simulink model "heli_q8_final"  (R2020b)
settings: Solver=ode1  StartTime=0.0  StopTime=inf  FixedStep=0.002  RelTol=1e-3  EnableMultiTasking=on
PostLoadFcn:
  | qc_set_target_type(getConfigSet(bdroot, 'QUARC Default Target Configuration'));
undefined symbols (not defined in the file or in its folder): A_d, A_obs, B_d, B_obs, C, C_d, elevation_offset, F, HIL, Joystick_gain_x, Joystick_gain_y, K, Kpd, Kpp, L, Q_d, qc_get_step_size, R_flying, V_s0
libraries: quarc_library x34, simulink x7, pid_lib x1
(part 1 of 2)
settings Model: SimulationMode=external  ExtModeTrigDuration=600000  Creator=Rchan  LastModifiedBy=wiktorjr
settings SolverCC: PositivePriorityOrder=on
settings DataIOCC: LimitDataPoints=on  SaveFormat=Array  SignalLoggingSaveFormat=ModelDataLogs  ReturnWorkspaceOutputs=off
settings OptimizationCC: ExpressionDepthLimit=2147483647  InitFltsAndDblsToZero=on  LifeSpan=inf
settings DebuggingCC: SaveWithParameterizedLinksMsg=none  UnderspecifiedInitializationDetection=Classic  MergeDetectMultiDrivingBlocksExec=none  SolverPrmCheckMsg=warning  MultiTaskDSMMsg=warning  MultiTaskCondExecSysMsg=none  FcnCallInpInsideContextMsg=warning  AllowSymbolicDim=off  StateNameClashWarn=warning  SFUnexpectedBacktrackingDiag=warning  SFNoUnconditionalDefaultTransitionDiag=warning  SFExecutionAtInitializationDiag=none  ArithmeticOperatorsInVariantConditions=warning
settings HardwareCC: ProdBitPerPointer=32  ProdBitPerSizeT=32  ProdBitPerPtrDiffT=32  ProdLargestAtomicFloat=None  ProdIntDivRoundTo=Undefined  ProdEndianess=Unspecified  ProdWordSize=32  ProdHWDeviceType=32-bit Generic
settings ModelReferenceCC: PropagateSignalLabelsOutOfModel=off
settings SFSimCC: SimUseLocalCustomCode=off  CustomCodeUndefinedFunction=UseInterfaceOnly
settings RTWCC: Description=QUARC Win64 Target  SystemTargetFile=quarc_win64.tlc  TemplateMakefile=quarc_default_tmf  RTWUseLocalCustomCode=off
settings CodeAppCC: StateflowObjectComments=on
settings GRTTargetCC: TargetLangStandard=C89/C90 (ANSI)  ParMdlRefBuildCompliant=off  CompOptLevelCompliant=off  CombineOutputUpdateFcns=off  MatFileLogging=off  GRTInterface=on  UseToolchainInfoCompliant=off  ExtMode=on  ExtModeMexFile=quarc_comm
settings ConfigComp: CovMetricSettings=dw  CovSaveCumulativeToWorkspaceVar=on  CovSaveSingleToWorkspaceVar=on  CovExternalEMLEnable=off  CovSFcnEnable=off

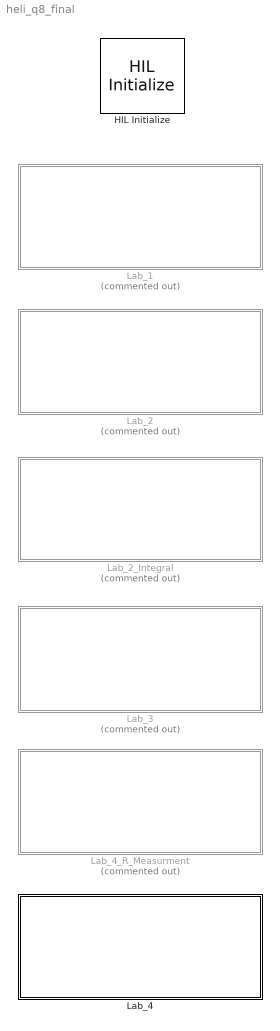
== system heli_q8_final ==
  HIL Initialize : quarc_library/Data Acquisition/Generic/Configuration/HIL Initialize  Priority=-99  object_name=HIL-1  board_type=q8_usb  board_number=0  board_options=update_rate=normal;decimation=1  exclusive=off  active=off  hardware_clocks=[0:2]  clock_modes=[]  initial_clock_frequencies=[]  set_clock_params_at_start=off  set_clock_params_at_switch_in=off  set_clock_frequencies_at_start=off  set_clock_frequencies_at_switch_in=off  analog_input_channels=[0:7]  analog_input_configurations=[]  analog_input_maximums=10  analog_input_minimums=-10  set_analog_input_params_at_start=on  set_analog_input_params_at_switch_in=off  analog_output_channels=[0:7]  analog_output_maximums=10  analog_output_minimums=-10  initial_analog_outputs=[0]  final_analog_outputs=[0]  watchdog_analog_outputs=0  set_analog_output_params_at_start=on  set_analog_output_params_at_switch_in=off  set_analog_outputs_at_start=on  set_analog_outputs_at_switch_in=off  set_analog_outputs_at_terminate=on  set_analog_outputs_at_switch_out=off  set_analog_outputs_on_watchdog=off  digital_input_channels=[]  digital_output_channels=[]  digital_output_configuration=[]  initial_digital_outputs=[1]  final_digital_outputs=[1]  watchdog_digital_outputs=[1]  set_digital_output_params_at_start=off  set_digital_output_params_at_switch_in=off  set_digital_outputs_at_start=on  set_digital_outputs_at_switch_in=off  set_digital_outputs_at_terminate=on  set_digital_outputs_at_switch_out=off  set_digital_outputs_on_watchdog=off  encoder_channels=[0:7]  quadrature=[4]  encoder_filter_frequency=[]  initial_encoder_counts=[0]  set_encoder_params_at_start=on  set_encoder_params_at_switch_in=off  set_encoder_counts_at_start=on  set_encoder_counts_at_switch_in=off  pwm_channels=[0:7]  pwm_modes=0  pwm_frequency=99.532799999999995e6/4095  pwm_configuration=[0]  pwm_alignment=[0]  pwm_polarity=[1]  pwm_leading_deadband=[0]  pwm_trailing_deadband=[0]  initial_pwm_outputs=[0]  final_pwm_outputs=[0]  watchdog_pwm_outputs=[0]  set_pwm_params_at_start=on  set_pwm_params_at_switch_in=off  set_pwm_outputs_at_start=on  set_pwm_outputs_at_switch_in=off  set_pwm_outputs_at_terminate=on  set_pwm_outputs_at_switch_out=off  set_pwm_outputs_on_watchdog=off  other_output_channels=[]  initial_other_outputs=[]  final_other_outputs=[]  watchdog_other_outputs=[]  set_other_outputs_at_start=off  set_other_outputs_at_switch_in=off  set_other_outputs_at_terminate=off  set_other_outputs_at_switch_out=off  set_other_outputs_on_watchdog=off
  Lab_1 : Subsystem  Commented=on
  Lab_2 : Subsystem  Commented=on
  Lab_2_Integral : Subsystem  Commented=on
  Lab_3 : Subsystem  Commented=on
  Lab_4 : Subsystem
  Lab_4_R_Measurment : Subsystem  Commented=on

== system heli_q8_final/Lab_1 ==
  note: Pitch test signal
  note: Elevation test signal
  Constant2 : Constant  Value=0
  Constant3 : Constant  Value=0.5
  Conversion : Subsystem
  Demux : Demux  Outputs=6
  Demux1 : Demux  Outputs=8
  Elevation controller : Subsystem
  Heli 3D : Subsystem
  Joystick : Subsystem
  Manual Switch2 : ManualSwitch
  Manual Switch3 : ManualSwitch  CurrentSetting=0
  Mux : Mux  Inputs=6
  Mux1 : Mux  Inputs=3
  Pitch controller : Subsystem
  Pulse Generator : DiscretePulseGenerator  PulseType=Time based  Amplitude=-1  Period=40  PulseWidth=50
  Ramp1 : simulink/Sources/Ramp  slope=0.05  start=0  InitialOutput=-0.5
  Ramp3 : simulink/Sources/Ramp  slope=0.1  start=45  InitialOutput=0
  Saturation : Saturate  UpperLimit=0
  Saturation2 : Saturate  LowerLimit=0
  Scope : Scope  NumInputPorts=4
  Step1 : Step  Time=15  SampleTime=0
  Step4 : Step  Time=40  SampleTime=0
  Sum1 : Sum  Inputs=+-|
  Sum4 : Sum  Inputs=+|-
  Sum5 : Sum  Inputs=+|+
  Switch : Switch  Criteria=u2 > Threshold
  To File : ToFile  Filename=Test.mat
  wires:
  Demux/4 -> Pitch controller/3(p~dot [rad/s])  "p~dot"
  Mux/1 -> Mux1/1, Demux/1
  Manual Switch2/1 -> Mux1/2, Pitch controller/1(p~c [rad])  "p_c"
  Elevation controller/1(V~s [V]) -> Conversion/2(Vs [V])
  Heli 3D/2(Travel rate [rad/s]) -> Mux/2  "lambda~_dot"
  Pitch controller/1(V~d [V]) -> Conversion/1(Vd [V])
  Heli 3D/6(Elevation rate [rad/s]) -> Mux/6  "e~dot"
  Demux/3 -> Pitch controller/2(p~ [rad])  "p~"
  Demux/6 -> Elevation controller/2(e~dot [rad/s])  "e~dot"
  Heli 3D/1(Travel [rad]) -> Mux/1  "lambda~"
  Conversion/2(Vb [V]) -> Heli 3D/2(Vb [V])
  Demux/5 -> Elevation controller/1(e~ [rad])  "e~"
  Heli 3D/5(Elevation [rad]) -> Mux/5  "e~"
  Heli 3D/3(Pitch [rad]) -> Mux/3  "p~"
  Heli 3D/4(Pitch rate [rad/s]) -> Mux/4  "p~dot"
  Conversion/1(Vf [V]) -> Heli 3D/1(Vf [V])
  Sum1/1 -> Manual Switch3/2
  Manual Switch3/1 -> Mux1/3, Elevation controller/3(e~c [rad])  "e_c"
  Sum5/1 -> Switch/1
  Joystick/2(Y) -> Manual Switch3/1  "e_c"
  Sum4/1 -> Switch/2
  Step4/1 -> Sum4/2
  Step1/1 -> Sum4/1
  Constant3/1 -> Sum5/2
  Joystick/1(X) -> Manual Switch2/2  "p_c"
  Switch/1 -> Manual Switch2/1
  Pulse Generator/1 -> Sum5/1
  Constant2/1 -> Switch/3
  Mux1/1 -> Demux1/1, To File/1
  Demux1/7 -> Scope/3  "p_c"
  Demux1/8 -> Scope/4  "e_c"
  Demux1/3 -> Scope/1  "p~"
  Demux1/5 -> Scope/2  "e~"
  Ramp1/1 -> Saturation/1
  Ramp3/1 -> Saturation2/1
  Saturation/1 -> Sum1/1
  Saturation2/1 -> Sum1/2

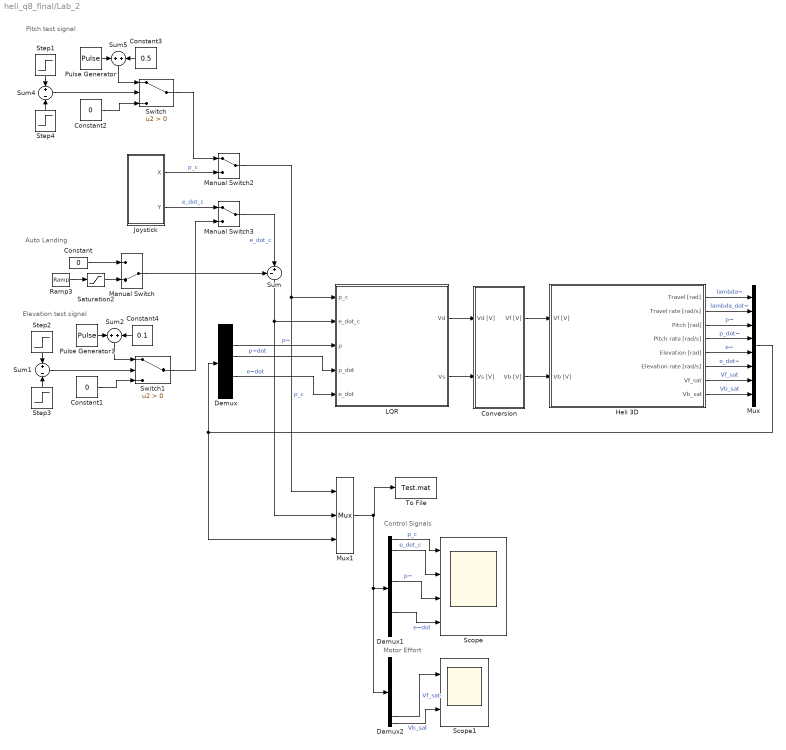
== system heli_q8_final/Lab_2 ==
  note: Auto Landing
  note: Motor Effort
  note: Control Signals
  note: Elevation test signal
  note: Pitch test signal
  Constant : Constant  Value=0
  Constant1 : Constant  Value=0
  Constant2 : Constant  Value=0
  Constant3 : Constant  Value=0.5
  Constant4 : Constant  Value=0.1
  Conversion : Subsystem
  Demux : Demux  Outputs=8
  Demux1 : Demux  Outputs=10
  Demux2 : Demux  Outputs=10
  Heli 3D : Subsystem
  Joystick : Subsystem
  LQR : Subsystem
  Manual Switch : ManualSwitch  CurrentSetting=0
  Manual Switch2 : ManualSwitch
  Manual Switch3 : ManualSwitch
  Mux : Mux  Inputs=8
  Mux1 : Mux  Inputs=3
  Pulse Generator : DiscretePulseGenerator  PulseType=Time based  Amplitude=-1  Period=15  PulseWidth=50
  Pulse Generator1 : DiscretePulseGenerator  PulseType=Time based  Amplitude=-0.2  Period=10  PulseWidth=50
  Ramp3 : simulink/Sources/Ramp  slope=0.15  start=45  InitialOutput=0
  Saturation2 : Saturate  UpperLimit=1  LowerLimit=0
  Scope : Scope  NumInputPorts=4
  Scope1 : Scope  NumInputPorts=2
  Step1 : Step  Time=15  SampleTime=0
  Step2 : Step  Time=15  SampleTime=0
  Step3 : Step  Time=40  SampleTime=0
  Step4 : Step  Time=40  SampleTime=0
  Sum : Sum  Inputs=-+|
  Sum1 : Sum  Inputs=+|-
  Sum2 : Sum  Inputs=+|+
  Sum4 : Sum  Inputs=+|-
  Sum5 : Sum  Inputs=+|+
  Switch : Switch  Criteria=u2 > Threshold
  Switch1 : Switch  Criteria=u2 > Threshold
  To File : ToFile  Filename=Test.mat
  wires:
  Heli 3D/4(Pitch rate [rad/s]) -> Mux/4  "p_dot~"
  Demux/6 -> LQR/5(e_dot)  "e~dot"
  Demux/3 -> LQR/3(p)  "p~"
  Heli 3D/3(Pitch [rad]) -> Mux/3  "p~"
  Manual Switch2/1 -> LQR/1(p_c), Mux1/1  "p_c"
  Manual Switch3/1 -> Sum/2  "e_dot_c"
  Mux/1 -> Mux1/3, Demux/1
  Demux/4 -> LQR/4(p_dot)  "p~dot"
  Heli 3D/5(Elevation [rad]) -> Mux/5  "e~"
  Conversion/1(Vf [V]) -> Heli 3D/1(Vf [V])
  Heli 3D/6(Elevation rate [rad/s]) -> Mux/6  "e_dot~"
  Heli 3D/1(Travel [rad]) -> Mux/1  "lambda~"
  Heli 3D/2(Travel rate [rad/s]) -> Mux/2  "lambda_dot~"
  Conversion/2(Vb [V]) -> Heli 3D/2(Vb [V])
  LQR/1(Vd) -> Conversion/1(Vd [V])
  LQR/2(Vs) -> Conversion/2(Vs [V])
  Joystick/1(X) -> Manual Switch2/2  "p_c"
  Step4/1 -> Sum4/2
  Pulse Generator/1 -> Sum5/1
  Constant3/1 -> Sum5/2
  Sum4/1 -> Switch/2
  Sum5/1 -> Switch/1
  Step1/1 -> Sum4/1
  Constant2/1 -> Switch/3
  Switch/1 -> Manual Switch2/1
  Joystick/2(Y) -> Manual Switch3/1  "e_dot_c"
  Heli 3D/7(Vf_sat) -> Mux/7  "Vf_sat"
  Heli 3D/8(Vb_sat) -> Mux/8  "Vb_sat"
  Mux1/1 -> Demux2/1, Demux1/1, To File/1
  Demux1/1 -> Scope/1  "p_c"
  Demux1/2 -> Scope/2  "e_dot_c"
  Demux1/5 -> Scope/3  "p~"
  Demux1/8 -> Scope/4  "e~dot"
  Demux2/9 -> Scope1/1  "Vf_sat"
  Demux2/10 -> Scope1/2  "Vb_sat"
  Step2/1 -> Sum1/1
  Sum2/1 -> Switch1/1
  Constant1/1 -> Switch1/3
  Pulse Generator1/1 -> Sum2/1
  Constant4/1 -> Sum2/2
  Step3/1 -> Sum1/2
  Sum1/1 -> Switch1/2
  Ramp3/1 -> Saturation2/1
  Switch1/1 -> Manual Switch3/2
  Saturation2/1 -> Manual Switch/2
  Constant/1 -> Manual Switch/1
  Manual Switch/1 -> Sum/1
  Sum/1 -> Mux1/2, LQR/2(e_dot_c)

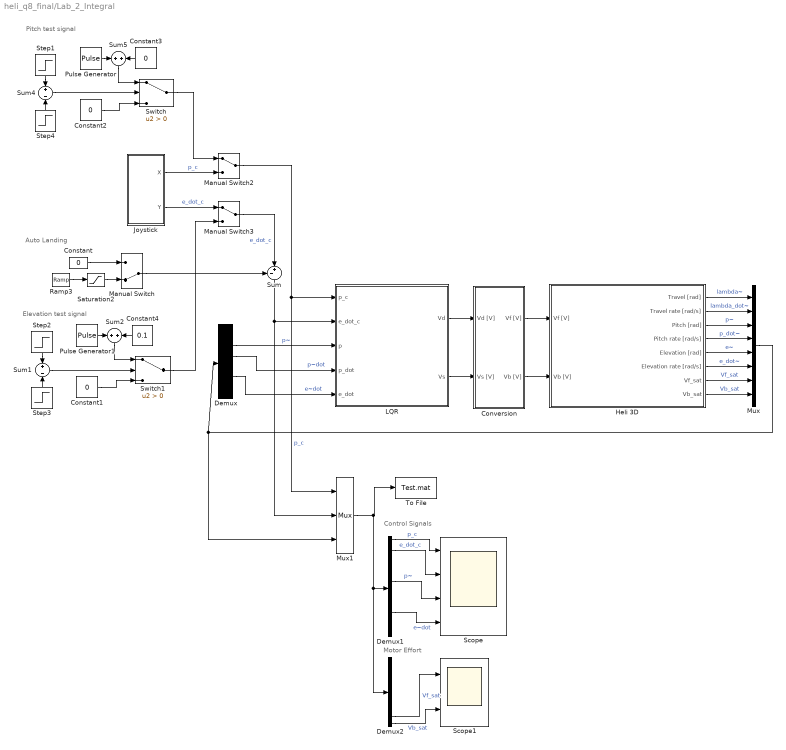
== system heli_q8_final/Lab_2_Integral ==
  note: Auto Landing
  note: Elevation test signal
  note: Motor Effort
  note: Pitch test signal
  note: Control Signals
  Constant{,1..3} (4 alike) : Constant  Value=0
  Constant4 : Constant  Value=0.1
  Conversion : Subsystem
  Demux : Demux  Outputs=8
  Demux1 : Demux  Outputs=10
  Demux2 : Demux  Outputs=10
  Heli 3D : Subsystem
  Joystick : Subsystem
  LQR : Subsystem
  Manual Switch : ManualSwitch  CurrentSetting=0
  Manual Switch2 : ManualSwitch
  Manual Switch3 : ManualSwitch
  Mux : Mux  Inputs=8
  Mux1 : Mux  Inputs=3
  Pulse Generator : DiscretePulseGenerator  PulseType=Time based  Amplitude=-0.5  Period=15  PulseWidth=50  PhaseDelay=-10
  Pulse Generator1 : DiscretePulseGenerator  PulseType=Time based  Amplitude=-0.2  Period=10  PulseWidth=50
  Ramp3 : simulink/Sources/Ramp  slope=0.15  start=45  InitialOutput=0
  Saturation2 : Saturate  UpperLimit=1  LowerLimit=0
  Scope : Scope  NumInputPorts=4
  Scope1 : Scope  NumInputPorts=2
  Step1 : Step  Time=15  SampleTime=0
  Step2 : Step  Time=15  SampleTime=0
  Step3 : Step  Time=40  SampleTime=0
  Step4 : Step  Time=40  SampleTime=0
  Sum : Sum  Inputs=-+|
  Sum1 : Sum  Inputs=+|-
  Sum2 : Sum  Inputs=+|+
  Sum4 : Sum  Inputs=+|-
  Sum5 : Sum  Inputs=+|+
  Switch : Switch  Criteria=u2 > Threshold
  Switch1 : Switch  Criteria=u2 > Threshold
  To File : ToFile  Filename=Test.mat
  wires:
  Sum/1 -> Mux1/2, LQR/2(e_dot_c)
  Constant4/1 -> Sum2/2
  Ramp3/1 -> Saturation2/1
  Constant2/1 -> Switch/3
  Demux/3 -> LQR/3(p)  "p~"
  Step3/1 -> Sum1/2
  Demux1/1 -> Scope/1  "p_c"
  Switch1/1 -> Manual Switch3/2
  Constant/1 -> Manual Switch/1
  Heli 3D/5(Elevation [rad]) -> Mux/5  "e~"
  Mux/1 -> Mux1/3, Demux/1
  Demux1/2 -> Scope/2  "e_dot_c"
  Demux1/8 -> Scope/4  "e~dot"
  Demux2/9 -> Scope1/1  "Vf_sat"
  Demux2/10 -> Scope1/2  "Vb_sat"
  Sum1/1 -> Switch1/2
  Sum4/1 -> Switch/2
  Pulse Generator1/1 -> Sum2/1
  Manual Switch/1 -> Sum/1
  Heli 3D/4(Pitch rate [rad/s]) -> Mux/4  "p_dot~"
  Heli 3D/8(Vb_sat) -> Mux/8  "Vb_sat"
  Constant1/1 -> Switch1/3
  Step2/1 -> Sum1/1
  Switch/1 -> Manual Switch2/1
  LQR/2(Vs) -> Conversion/2(Vs [V])
  Step4/1 -> Sum4/2
  Pulse Generator/1 -> Sum5/1
  Manual Switch2/1 -> Mux1/1, LQR/1(p_c)  "p_c"
  Saturation2/1 -> Manual Switch/2
  Mux1/1 -> Demux2/1, Demux1/1, To File/1
  Demux1/5 -> Scope/3  "p~"
  Constant3/1 -> Sum5/2
  Sum2/1 -> Switch1/1
  Heli 3D/2(Travel rate [rad/s]) -> Mux/2  "lambda_dot~"
  Sum5/1 -> Switch/1
  Manual Switch3/1 -> Sum/2  "e_dot_c"
  Step1/1 -> Sum4/1
  Heli 3D/1(Travel [rad]) -> Mux/1  "lambda~"
  Joystick/1(X) -> Manual Switch2/2  "p_c"
  Demux/4 -> LQR/4(p_dot)  "p~dot"
  Joystick/2(Y) -> Manual Switch3/1  "e_dot_c"
  Heli 3D/7(Vf_sat) -> Mux/7  "Vf_sat"
  LQR/1(Vd) -> Conversion/1(Vd [V])
  Heli 3D/6(Elevation rate [rad/s]) -> Mux/6  "e_dot~"
  Heli 3D/3(Pitch [rad]) -> Mux/3  "p~"
  Demux/6 -> LQR/5(e_dot)  "e~dot"
  Conversion/2(Vb [V]) -> Heli 3D/2(Vb [V])
  Conversion/1(Vf [V]) -> Heli 3D/1(Vf [V])

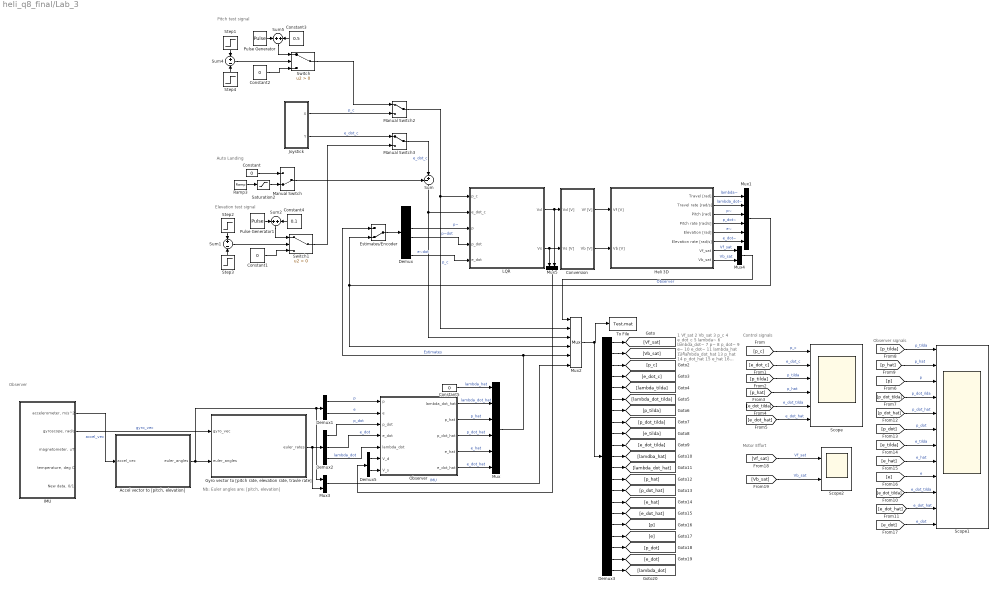
== system heli_q8_final/Lab_3 ==
  note: Motor Effort
  note: Control signals
  note: 1   Vf_sat
      | 2   Vb_sat
      | 3   p_c
      | 4   e_dot_c
      | 5   lambda~
      | 6   lambda_dot~
      | 7   p~
      | 8   p_dot~
      | 9   e~
      | 10 e_dot~
      | 11 lambda_hat
      | 12 lambda_dot_hat
      | 13 p_hat
      | 14 p_dot_hat
      | 15 e_hat
      | 16 e_dot_hat
      | 17 p
      | 18 e
      | 19 p_dot
      | 20 e_dot
      | 21 lambda_dot
  note: Observer
  note: Nb: Euler angles are: [pitch, elevation]
  note: Pitch test signal
  note: Elevation test signal
  note: Auto Landing
  note: Observer signals
  "Accel vector to [pitch, elevation]" : MATLAB Function  TreatAsAtomicUnit=on
  Constant{,1..2,5} (4 alike) : Constant  Value=0
  Constant3 : Constant  Value=0.5
  Constant4 : Constant  Value=0.1
  Conversion : Subsystem
  Demux : Demux  Outputs=6
  Demux1 : Demux  Outputs=2
  Demux2 : Demux  Outputs=3
  Demux3 : Demux  Outputs=21
  Demux5 : Demux  Outputs=2
  Estimates/Encoder : ManualSwitch  CurrentSetting=0
  "Gyro vector to [pitch rate, elevation rate, travle rate]" : MATLAB Function  TreatAsAtomicUnit=on
  Heli 3D : Subsystem
  IMU : Subsystem
  Joystick : Subsystem
  LQR : Subsystem
  Manual Switch : ManualSwitch  CurrentSetting=0
  Manual Switch2 : ManualSwitch
  Manual Switch3 : ManualSwitch
  Mux : Mux  Inputs=6
  Mux1 : Mux  Inputs=6
  Mux2 : Mux  Inputs=6
  Mux3 : Mux  Inputs=2
  Mux4 : Mux  Inputs=2
  Mux5 : Mux  Inputs=2
  Observer : Subsystem
  Pulse Generator : DiscretePulseGenerator  PulseType=Time based  Amplitude=-1  Period=15  PulseWidth=50  PhaseDelay=-10
  Pulse Generator1 : DiscretePulseGenerator  PulseType=Time based  Amplitude=-0.2  Period=10  PulseWidth=50
  Ramp3 : simulink/Sources/Ramp  slope=0.15  start=45  InitialOutput=0
  Saturation2 : Saturate  UpperLimit=1  LowerLimit=0
  Scope : Scope  NumInputPorts=6
  Scope1 : Scope  NumInputPorts=12
  Scope2 : Scope  NumInputPorts=2
  Step1 : Step  Time=15  SampleTime=0
  Step2 : Step  Time=15  SampleTime=0
  Step3 : Step  Time=40  SampleTime=0
  Step4 : Step  Time=40  SampleTime=0
  Sum : Sum  Inputs=-+|
  Sum1 : Sum  Inputs=+|-
  Sum2 : Sum  Inputs=+|+
  Sum4 : Sum  Inputs=+|-
  Sum5 : Sum  Inputs=+|+
  Switch : Switch  Criteria=u2 > Threshold
  Switch1 : Switch  Criteria=u2 > Threshold
  To File : ToFile  Filename=Test.mat
  wires:
  Demux2/1 -> Observer/3(p_dot)  "p_dot"
  "Gyro vector to [pitch rate, elevation rate, travle rate]"/1(euler_rates) -> Mux3/2, Demux2/1
  "Accel vector to [pitch, elevation]"/1(euler_angles) -> Mux3/1, Demux1/1, "Gyro vector to [pitch rate, elevation rate, travle rate]"/2(euler_angles)
  Demux2/2 -> Observer/4(e_dot)  "e_dot"
  Demux2/3 -> Observer/5(lambda_dot)  "lambda_dot"
  Demux1/2 -> Observer/2(e)  "e"
  IMU/2("gyroscope, rad/s") -> "Gyro vector to [pitch rate, elevation rate, travle rate]"/1(gyro_vec)  "gyro_vec"
  Demux1/1 -> Observer/1(p)  "p"
  IMU/1("accelerometer, m/s^2") -> "Accel vector to [pitch, elevation]"/1(accel_vec)  "accel_vec"
  Step3/1 -> Sum1/2
  Heli 3D/3(Pitch [rad]) -> Mux1/3  "p~"
  Heli 3D/7(Vf_sat) -> Mux4/1  "Vf_sat"
  Joystick/1(X) -> Manual Switch2/2  "p_c"
  Constant3/1 -> Sum5/2
  Sum5/1 -> Switch/1
  Manual Switch3/1 -> Sum/2  "e_dot_c"
  Sum2/1 -> Switch1/1
  Saturation2/1 -> Manual Switch/2
  Mux2/1 -> Demux3/1, To File/1
  Manual Switch2/1 -> Mux2/2, LQR/1(p_c)  "p_c"
  Pulse Generator/1 -> Sum5/1
  Step1/1 -> Sum4/1
  Step4/1 -> Sum4/2
  Heli 3D/4(Pitch rate [rad/s]) -> Mux1/4  "p_dot~"
  Step2/1 -> Sum1/1
  Constant1/1 -> Switch1/3
  Pulse Generator1/1 -> Sum2/1
  Heli 3D/1(Travel [rad]) -> Mux1/1  "lambda~"
  Switch/1 -> Manual Switch2/1
  Sum4/1 -> Switch/2
  Manual Switch/1 -> Sum/1
  Mux1/1 -> Estimates/Encoder/2, Mux2/4  "Observer"
  Heli 3D/2(Travel rate [rad/s]) -> Mux1/2  "lambda_dot~"
  Switch1/1 -> Manual Switch3/2
  Conversion/2(Vb [V]) -> Heli 3D/2(Vb [V])
  Heli 3D/5(Elevation [rad]) -> Mux1/5  "e~"
  Demux/3 -> LQR/3(p)  "p~"
  Constant4/1 -> Sum2/2
  Constant2/1 -> Switch/3
  Ramp3/1 -> Saturation2/1
  Sum/1 -> Mux2/3, LQR/2(e_dot_c)
  Heli 3D/8(Vb_sat) -> Mux4/2  "Vb_sat"
  Joystick/2(Y) -> Manual Switch3/1  "e_dot_c"
  LQR/2(Vs) -> Conversion/2(Vs [V]), Mux5/1
  Constant/1 -> Manual Switch/1
  Sum1/1 -> Switch1/2
  Heli 3D/6(Elevation rate [rad/s]) -> Mux1/6  "e_dot~"
  Demux/6 -> LQR/5(e_dot)  "e~dot"
  Demux/4 -> LQR/4(p_dot)  "p~dot"
  LQR/1(Vd) -> Conversion/1(Vd [V]), Mux5/2
  Conversion/1(Vf [V]) -> Heli 3D/1(Vf [V])
  Mux/1 -> Estimates/Encoder/1, Mux2/5  "Estimates"
  Mux3/1 -> Mux2/6  "IMU"
  Mux4/1 -> Mux2/1
  Constant5/1 -> Mux/1  "lambda_hat"
  Observer/1(lambda_dot_hat) -> Mux/2  "lambda_dot_hat"
  Observer/2(p_hat) -> Mux/3  "p_hat"
  Observer/3(p_dot_hat) -> Mux/4  "p_dot_hat"
  Observer/4(e_hat) -> Mux/5  "e_hat"
  Observer/5(e_dot_hat) -> Mux/6  "e_dot_hat"
  Estimates/Encoder/1 -> Demux/1
  Demux5/1 -> Observer/6(V_d)
  Demux5/2 -> Observer/7(V_s)
  Mux5/1 -> Demux5/1
  Demux3/1 -> [Vf_sat]
  Demux3/2 -> [Vb_sat]
  Demux3/3 -> [p_c]
  Demux3/4 -> [e_dot_c]
  Demux3/5 -> [lambda_tilda]
  Demux3/6 -> [lambda_dot_tilda]
  Demux3/7 -> [p_tilda]
  Demux3/8 -> [p_dot_tilda]
  Demux3/9 -> [e_tilda]
  Demux3/10 -> [e_dot_tilda]
  Demux3/11 -> [lamdba_hat]
  Demux3/12 -> [lambda_dot_hat]
  Demux3/13 -> [p_hat]
  Demux3/14 -> [p_dot_hat]
  Demux3/15 -> [e_hat]
  Demux3/16 -> [e_dot_hat]
  Demux3/17 -> [p]
  Demux3/18 -> [e]
  Demux3/19 -> [p_dot]
  Demux3/20 -> [e_dot]
  Demux3/21 -> [lambda_dot]
  [p_c] -> Scope/1  "p_c"
  [e_dot_c] -> Scope/2  "e_dot_c"
  [p_tilda] -> Scope/3  "p_tilda"
  [p_hat] -> Scope/4  "p_hat"
  [e_dot_tilda] -> Scope/5  "e_dot_tilda"
  [e_dot_hat] -> Scope/6  "e_dot_hat"
  [p_hat] -> Scope1/2  "p_hat"
  [e_dot_hat] -> Scope1/11  "e_dot_hat"
  [e_dot_tilda] -> Scope1/10  "e_dot_tilda"
  [p_tilda] -> Scope1/1  "p_tilda"
  [p] -> Scope1/3  "p"
  [p_dot_tilda] -> Scope1/4  "p_dot_ilda"
  [p_dot_hat] -> Scope1/5  "p_dot_hat"
  [p_dot] -> Scope1/6  "p_dot"
  [e_tilda] -> Scope1/7  "e_tilda"
  [e_hat] -> Scope1/8  "e_hat"
  [e] -> Scope1/9  "e"
  [e_dot] -> Scope1/12  "e_dot"
  [Vf_sat] -> Scope2/1  "Vf_sat"
  [Vb_sat] -> Scope2/2  "Vb_sat"

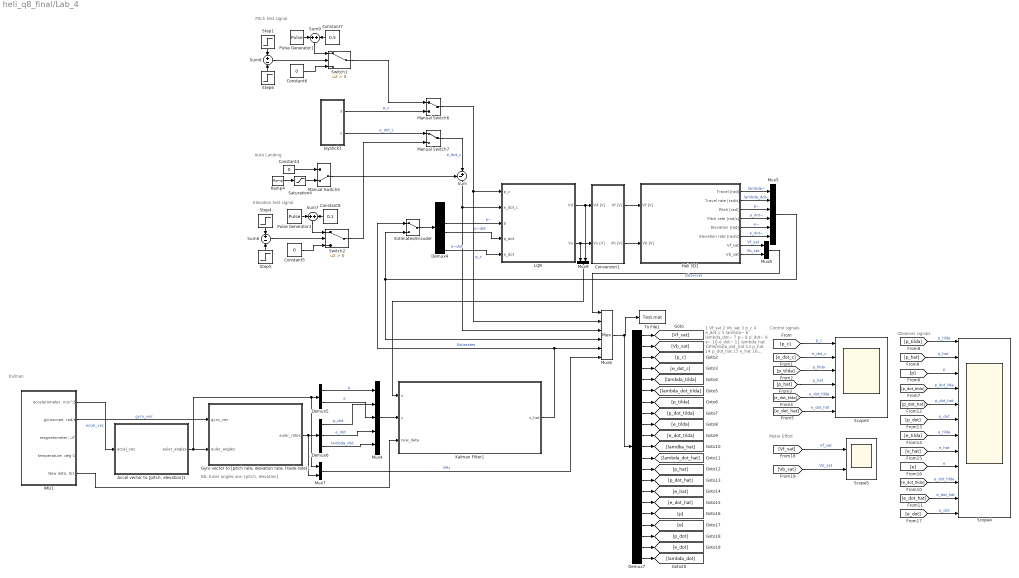
== system heli_q8_final/Lab_4 ==
  note: Control signals
  note: 1   Vf_sat
      | 2   Vb_sat
      | 3   p_c
      | 4   e_dot_c
      | 5   lambda~
      | 6   lambda_dot~
      | 7   p~
      | 8   p_dot~
      | 9   e~
      | 10 e_dot~
      | 11 lambda_hat
      | 12 lambda_dot_hat
      | 13 p_hat
      | 14 p_dot_hat
      | 15 e_hat
      | 16 e_dot_hat
      | 17 p
      | 18 e
      | 19 p_dot
      | 20 e_dot
      | 21 lambda_dot
  note: Elevation test signal
  note: Kalman
  note: Auto Landing
  note: Nb: Euler angles are: [pitch, elevation]
  note: Observer signals
  note: Pitch test signal
  note: Motor Effort
  "Accel vector to [pitch, elevation]1" : MATLAB Function  TreatAsAtomicUnit=on
  Constant4 : Constant  Value=0
  Constant5 : Constant  Value=0
  Constant6 : Constant  Value=0
  Constant7 : Constant  Value=0.5
  Constant8 : Constant  Value=0.1
  Conversion1 : Subsystem
  Demux4 : Demux  Outputs=6
  Demux5 : Demux  Outputs=2
  Demux6 : Demux  Outputs=3
  Demux7 : Demux  Outputs=21
  Estimates/Encoder : ManualSwitch
  "Gyro vector to [pitch rate, elevation rate, travle rate]1" : MATLAB Function  TreatAsAtomicUnit=on
  Heli 3D1 : Subsystem
  IMU1 : Subsystem
  Joystick1 : Subsystem
  Kalman Filter1 : Subsystem
  LQR : Subsystem
  Manual Switch5 : ManualSwitch  CurrentSetting=0
  Manual Switch6 : ManualSwitch
  Manual Switch7 : ManualSwitch
  Mux4 : Mux  Inputs=5
  Mux5 : Mux  Inputs=6
  Mux6 : Mux  Inputs=6
  Mux7 : Mux  Inputs=2
  Mux8 : Mux  Inputs=2
  Mux9 : Mux  Inputs=2
  Pulse Generator1 : DiscretePulseGenerator  PulseType=Time based  Amplitude=-1  Period=15  PulseWidth=50  PhaseDelay=-10
  Pulse Generator2 : DiscretePulseGenerator  PulseType=Time based  Amplitude=-0.2  Period=10  PulseWidth=50
  Ramp4 : simulink/Sources/Ramp  slope=0.15  start=45  InitialOutput=0
  Saturation4 : Saturate  UpperLimit=1  LowerLimit=0
  Scope3 : Scope  NumInputPorts=6
  Scope4 : Scope  NumInputPorts=12
  Scope5 : Scope  NumInputPorts=2
  Step1 : Step  Time=15  SampleTime=0
  Step4 : Step  Time=15  SampleTime=0
  Step5 : Step  Time=40  SampleTime=0
  Step6 : Step  Time=40  SampleTime=0
  Sum : Sum  Inputs=-+|
  Sum6 : Sum  Inputs=+|-
  Sum7 : Sum  Inputs=+|+
  Sum8 : Sum  Inputs=+|-
  Sum9 : Sum  Inputs=+|+
  Switch1 : Switch  Criteria=u2 > Threshold
  Switch2 : Switch  Criteria=u2 > Threshold
  To File1 : ToFile  Filename=Test.mat
  wires:
  Demux7/2 -> [Vb_sat]
  Demux7/12 -> [lambda_dot_hat]
  [e_dot] -> Scope4/12  "e_dot"
  [e_dot_hat] -> Scope4/11  "e_dot_hat"
  [p_c] -> Scope3/1  "p_c"
  Demux7/7 -> [p_tilda]
  Demux7/16 -> [e_dot_hat]
  Demux7/17 -> [p]
  Demux7/4 -> [e_dot_c]
  [p] -> Scope4/3  "p"
  [p_dot_hat] -> Scope4/5  "p_dot_hat"
  Heli 3D1/8(Vb_sat) -> Mux8/2  "Vb_sat"
  [p_hat] -> Scope4/2  "p_hat"
  [e_tilda] -> Scope4/7  "e_tilda"
  Demux7/14 -> [p_dot_hat]
  Demux7/15 -> [e_hat]
  [p_tilda] -> Scope4/1  "p_tilda"
  [e_hat] -> Scope4/8  "e_hat"
  Demux7/19 -> [p_dot]
  Demux7/13 -> [p_hat]
  Demux7/3 -> [p_c]
  Demux7/5 -> [lambda_tilda]
  Demux7/8 -> [p_dot_tilda]
  Demux7/21 -> [lambda_dot]
  Estimates/Encoder/1 -> Demux4/1
  Mux7/1 -> Mux6/6  "IMU"
  [e_dot_c] -> Scope3/2  "e_dot_c"
  [p_hat] -> Scope3/4  "p_hat"
  [p_dot_tilda] -> Scope4/4  "p_dot_ilda"
  [Vb_sat] -> Scope5/2  "Vb_sat"
  [Vf_sat] -> Scope5/1  "Vf_sat"
  Sum8/1 -> Switch1/2
  Switch1/1 -> Manual Switch6/1
  Heli 3D1/1(Travel [rad]) -> Mux5/1  "lambda~"
  Pulse Generator2/1 -> Sum7/1
  Constant5/1 -> Switch2/3
  Heli 3D1/4(Pitch rate [rad/s]) -> Mux5/4  "p_dot~"
  Step6/1 -> Sum8/2
  Step1/1 -> Sum8/1
  Manual Switch6/1 -> Mux6/2, LQR/1(p_c)  "p_c"
  Mux6/1 -> Demux7/1, To File1/1
  Pulse Generator1/1 -> Sum9/1
  Sum7/1 -> Switch2/1
  LQR/2(Vs) -> Conversion1/2(Vs [V]), Mux9/1
  Demux4/6 -> LQR/5(e_dot)  "e~dot"
  Heli 3D1/6(Elevation rate [rad/s]) -> Mux5/6  "e_dot~"
  Joystick1/2(Y) -> Manual Switch7/1  "e_dot_c"
  Demux4/3 -> LQR/3(p)  "p~"
  Constant6/1 -> Switch1/3
  Constant8/1 -> Sum7/2
  Demux4/4 -> LQR/4(p_dot)  "p~dot"
  Heli 3D1/5(Elevation [rad]) -> Mux5/5  "e~"
  Heli 3D1/2(Travel rate [rad/s]) -> Mux5/2  "lambda_dot~"
  Sum9/1 -> Switch1/1
  Manual Switch5/1 -> Sum/1
  Mux5/1 -> Estimates/Encoder/2, Mux6/4  "Observer"
  Joystick1/1(X) -> Manual Switch6/2  "p_c"
  Conversion1/2(Vb [V]) -> Heli 3D1/2(Vb [V])
  Constant4/1 -> Manual Switch5/1
  LQR/1(Vd) -> Conversion1/1(Vd [V]), Mux9/2
  Kalman Filter1/1(x_hat) -> Estimates/Encoder/1, Mux6/5  "Estimates"
  Conversion1/1(Vf [V]) -> Heli 3D1/1(Vf [V])
  [e_dot_hat] -> Scope3/6  "e_dot_hat"
  Demux7/18 -> [e]
  Demux7/9 -> [e_tilda]
  Sum6/1 -> Switch2/2
  Ramp4/1 -> Saturation4/1
  Sum/1 -> Mux6/3, LQR/2(e_dot_c)
  "Accel vector to [pitch, elevation]1"/1(euler_angles) -> Mux7/1, Demux5/1, "Gyro vector to [pitch rate, elevation rate, travle rate]1"/2(euler_angles)
  Switch2/1 -> Manual Switch7/2
  Demux5/2 -> Mux4/3  "e"
  IMU1/2("gyroscope, rad/s") -> "Gyro vector to [pitch rate, elevation rate, travle rate]1"/1(gyro_vec)  "gyro_vec"
  Manual Switch7/1 -> Sum/2  "e_dot_c"
  Saturation4/1 -> Manual Switch5/2
  [e_dot_tilda] -> Scope4/10  "e_dot_tilda"
  Demux6/3 -> Mux4/5  "lambda_dot"
  IMU1/1("accelerometer, m/s^2") -> "Accel vector to [pitch, elevation]1"/1(accel_vec)  "accel_vec"
  Heli 3D1/3(Pitch [rad]) -> Mux5/3  "p~"
  Demux6/2 -> Mux4/4  "e_dot"
  Demux7/20 -> [e_dot]
  "Gyro vector to [pitch rate, elevation rate, travle rate]1"/1(euler_rates) -> Mux7/2, Demux6/1
  Demux7/1 -> [Vf_sat]
  Step4/1 -> Sum6/1
  Demux7/6 -> [lambda_dot_tilda]
  [p_dot] -> Scope4/6  "p_dot"
  Demux6/1 -> Mux4/2  "p_dot"
  Demux7/11 -> [lamdba_hat]
  Demux5/1 -> Mux4/1  "p"
  [p_tilda] -> Scope3/3  "p_tilda"
  Heli 3D1/7(Vf_sat) -> Mux8/1  "Vf_sat"
  Mux9/1 -> Kalman Filter1/1(u)
  Constant7/1 -> Sum9/2
  [e] -> Scope4/9  "e"
  Step5/1 -> Sum6/2
  Mux8/1 -> Mux6/1
  [e_dot_tilda] -> Scope3/5  "e_dot_tilda"
  Demux7/10 -> [e_dot_tilda]
  IMU1/5("New data, 0/1") -> Kalman Filter1/3(new_data)
  Mux4/1 -> Kalman Filter1/2(y)

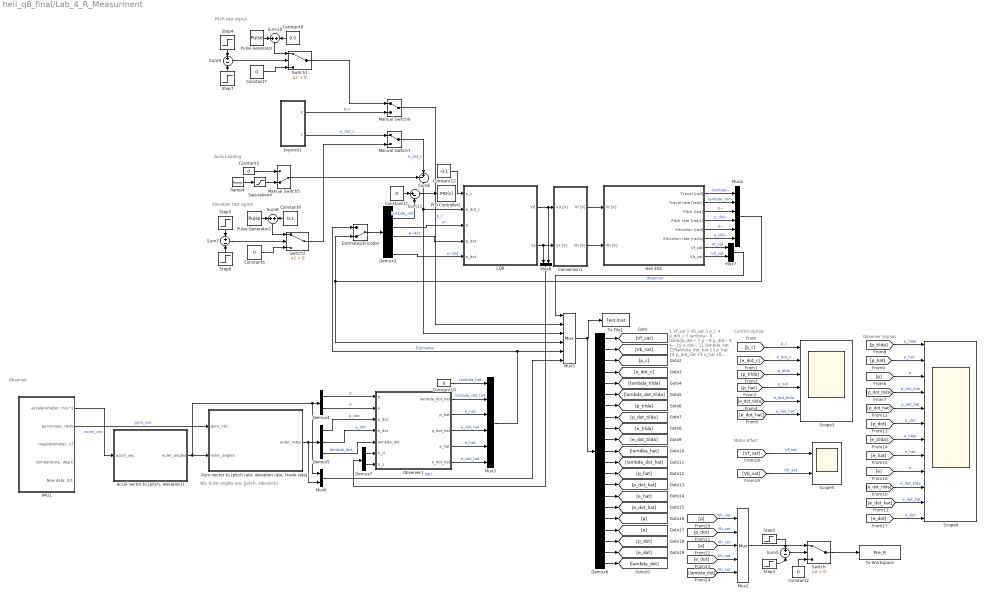
== system heli_q8_final/Lab_4_R_Measurment ==
  note: Control signals
  note: 1   Vf_sat
      | 2   Vb_sat
      | 3   p_c
      | 4   e_dot_c
      | 5   lambda~
      | 6   lambda_dot~
      | 7   p~
      | 8   p_dot~
      | 9   e~
      | 10 e_dot~
      | 11 lambda_hat
      | 12 lambda_dot_hat
      | 13 p_hat
      | 14 p_dot_hat
      | 15 e_hat
      | 16 e_dot_hat
      | 17 p
      | 18 e
      | 19 p_dot
      | 20 e_dot
      | 21 lambda_dot
  note: Elevation test signal
  note: Observer
  note: Auto Landing
  note: Nb: Euler angles are: [pitch, elevation]
  note: Observer signals
  note: Pitch test signal
  note: Motor Effort
  "Accel vector to [pitch, elevation]1" : MATLAB Function  TreatAsAtomicUnit=on
  Constant{2,5..7,10..11} (6 alike) : Constant  Value=0
  Constant12 : Constant  Value=-0.1
  Constant8 : Constant  Value=0.5
  Constant9 : Constant  Value=0.1
  Conversion1 : Subsystem
  Demux3 : Demux  Outputs=6
  Demux4 : Demux  Outputs=2
  Demux5 : Demux  Outputs=3
  Demux6 : Demux  Outputs=21
  Demux7 : Demux  Outputs=2
  Estimates/Encoder : ManualSwitch  CurrentSetting=0
  "Gyro vector to [pitch rate, elevation rate, travle rate]1" : MATLAB Function  TreatAsAtomicUnit=on
  Heli 3D1 : Subsystem
  IMU1 : Subsystem
  Joystick1 : Subsystem
  LQR : Subsystem
  Manual Switch5 : ManualSwitch  CurrentSetting=0
  Manual Switch6 : ManualSwitch
  Manual Switch7 : ManualSwitch
  Mux2 : Mux  Inputs=5
  Mux3 : Mux  Inputs=6
  Mux4 : Mux  Inputs=6
  Mux5 : Mux  Inputs=6
  Mux6 : Mux  Inputs=2
  Mux7 : Mux  Inputs=2
  Mux8 : Mux  Inputs=2
  Observer1 : Subsystem
  PID Controller1 : pid_lib/PID Controller  Controller=PID  Form=Parallel  TimeDomain=Continuous-time  UseExternalTs=off  SampleTime=-1  IntegratorMethod=Forward Euler  FilterMethod=Forward Euler  ControllerParametersSource=internal  P=0.8  I=0.2  D=0  UseFilter=on  N=100  TunerSelectOption=Transfer Function Based (PID Tuner App)  InitialConditionSource=internal  InitialConditionForIntegrator=0  InitialConditionForFilter=0  DifferentiatorICPrevScaledInput=0  ExternalReset=none  TrackingMode=off  Kt=1  LimitOutput=off  SatLimitsSource=internal  UpperSaturationLimit=inf  LowerSaturationLimit=-inf  LinearizeAsGain=on  AntiWindupMode=none  Kb=1  POutMin=[]  POutMax=[]  IOutMin=[]  IOutMax=[]  DOutMin=[]  DOutMax=[]  NOutMin=[]  NOutMax=[]  SumOutMin=[]  SumOutMax=[]  SaturationOutMin=[]  SaturationOutMax=[]  PParamMin=[]  PParamMax=[]  IParamMin=[]  IParamMax=[]  DParamMin=[]  DParamMax=[]  NParamMin=[]  NParamMax=[]  KbParamMin=[]  KbParamMax=[]  KtParamMin=[]  KtParamMax=[]  KbOutMin=[]  KbOutMax=[]  KtOutMin=[]  KtOutMax=[]  IntegratorOutMin=[]  IntegratorOutMax=[]  FilterOutMin=[]  FilterOutMax=[]  SumI1OutMin=[]  SumI1OutMax=[]  SumI2OutMin=[]  SumI2OutMax=[]  SumI3OutMin=[]  SumI3OutMax=[]  SumI4OutMin=[]  SumI4OutMax=[]  SumDOutMin=[]  SumDOutMax=[]  DifferentiatorOutMin=[]  DifferentiatorOutMax=[]  FilterDiffOutCoefMin=[]  FilterDiffOutCoefMax=[]  ReciprocalOutMin=[]  ReciprocalOutMax=[]  SumDenOutMin=[]  SumDenOutMax=[]  SumNumOutMin=[]  SumNumOutMax=[]  DivideOutMin=[]  DivideOutMax=[]  UdiffTsProdOutMin=[]  UdiffTsProdOutMax=[]  NTsProdOutMin=[]  NTsProdOutMax=[]  UintegralTsProdOutMin=[]  UintegralTsProdOutMax=[]  UngainTsProdOutMin=[]  UngainTsProdOutMax=[]  IntegratorContinuousStateAttributes=''  IntegratorStateMustResolveToSignalObject=off  IntegratorRTWStateStorageClass=Auto  FilterContinuousStateAttributes=''  FilterStateMustResolveToSignalObject=off  FilterRTWStateStorageClass=Auto  ParallelPVariant=InternalParameters  IdealPVariant=Disabled  IVariant=InternalParameters  DVariant=InternalParameters  IntegratorVariant=Continuous  SatVariant=Disabled  AWVariant=Passthrough  PCopyVariant=Disabled  TRVariant=Disabled  FdbkBlocksVariant=Forward  IdealPFdbkVariant=Disabled  SatFdbkVariant=Disabled  DerivativeFilterVariant=ContFilter  NVariant=InternalParameters  NCopyVariant=Disabled  FilterICVariant=InternalICsFilter  IntegratorICVariant=InternalICs  ExternalResetVariant=Disabled  TRSumVariant=Passthrough  SumFdbkVariant=Disabled  SumVariant=Sum_PID  TsampFilterVariant=InternalTs  TsampNgainVariant=Passthrough  TsampIntegralVariant=Passthrough  ExternalSaturationOutDataTypeStr=Inherit: Same as second input
  Pulse Generator : DiscretePulseGenerator  PulseType=Time based  Amplitude=-1  Period=15  PulseWidth=50  PhaseDelay=-10
  Pulse Generator1 : DiscretePulseGenerator  PulseType=Time based  Amplitude=-0.2  Period=10  PulseWidth=50
  Ramp4 : simulink/Sources/Ramp  slope=0.15  start=45  InitialOutput=0
  Saturation4 : Saturate  UpperLimit=1  LowerLimit=0
  Scope3 : Scope  NumInputPorts=6
  Scope4 : Scope  NumInputPorts=12
  Scope5 : Scope  NumInputPorts=2
  Step2 : Step  Time=40  SampleTime=0
  Step3 : Step  Time=50  After=2  SampleTime=0
  Step4 : Step  Time=15  SampleTime=0
  Step5 : Step  Time=15  SampleTime=0
  Step6 : Step  Time=40  SampleTime=0
  Step7 : Step  Time=40  SampleTime=0
  Sum10 : Sum  Inputs=+|+
  Sum11 : Sum  Inputs=|+-
  Sum5 : Sum  Inputs=+|-
  Sum6 : Sum  Inputs=-+|
  Sum7 : Sum  Inputs=+|-
  Sum8 : Sum  Inputs=+|+
  Sum9 : Sum  Inputs=+|-
  Switch : Switch  Criteria=u2 > Threshold
  Switch1 : Switch  Criteria=u2 > Threshold
  Switch2 : Switch  Criteria=u2 > Threshold
  To File1 : ToFile  Filename=Test.mat
  To Workspace : ToWorkspace  VariableName=Pre_R  SampleTime=-1
  wires:
  Sum5/1 -> Switch/2
  Mux2/1 -> Switch/1
  Step3/1 -> Sum5/2
  Constant2/1 -> Switch/3
  Step2/1 -> Sum5/1
  Switch/1 -> To Workspace/1
  Demux6/2 -> [Vb_sat]
  Demux6/12 -> [lambda_dot_hat]
  [e_dot] -> Scope4/12  "e_dot"
  [e_dot_hat] -> Scope4/11  "e_dot_hat"
  [p_c] -> Scope3/1  "p_c"
  Demux6/7 -> [p_tilda]
  Demux6/16 -> [e_dot_hat]
  Observer1/3(p_dot_hat) -> Mux3/4  "p_dot_hat"
  Demux6/17 -> [p]
  Demux6/4 -> [e_dot_c]
  [p] -> Scope4/3  "p"
  [p_dot_hat] -> Scope4/5  "p_dot_hat"
  Constant10/1 -> Mux3/1  "lambda_hat"
  Observer1/4(e_hat) -> Mux3/5  "e_hat"
  Observer1/2(p_hat) -> Mux3/3  "p_hat"
  Observer1/5(e_dot_hat) -> Mux3/6  "e_dot_hat"
  Heli 3D1/8(Vb_sat) -> Mux7/2  "Vb_sat"
  [p_hat] -> Scope4/2  "p_hat"
  [e_tilda] -> Scope4/7  "e_tilda"
  Demux6/14 -> [p_dot_hat]
  Demux6/15 -> [e_hat]
  [p_tilda] -> Scope4/1  "p_tilda"
  [e_hat] -> Scope4/8  "e_hat"
  Demux6/19 -> [p_dot]
  Demux6/13 -> [p_hat]
  Demux6/3 -> [p_c]
  Observer1/1(lambda_dot_hat) -> Mux3/2  "lambda_dot_hat"
  Demux6/5 -> [lambda_tilda]
  Demux6/8 -> [p_dot_tilda]
  Demux6/21 -> [lambda_dot]
  Estimates/Encoder/1 -> Demux3/1
  Mux6/1 -> Mux5/6  "IMU"
  [e_dot_c] -> Scope3/2  "e_dot_c"
  [p_hat] -> Scope3/4  "p_hat"
  [p_dot_tilda] -> Scope4/4  "p_dot_ilda"
  [Vb_sat] -> Scope5/2  "Vb_sat"
  [Vf_sat] -> Scope5/1  "Vf_sat"
  Sum9/1 -> Switch1/2
  Switch1/1 -> Manual Switch6/1
  Heli 3D1/1(Travel [rad]) -> Mux4/1  "lambda~"
  Pulse Generator1/1 -> Sum8/1
  Constant6/1 -> Switch2/3
  Heli 3D1/4(Pitch rate [rad/s]) -> Mux4/4  "p_dot~"
  Step7/1 -> Sum9/2
  Step4/1 -> Sum9/1
  Manual Switch6/1 -> Mux5/2  "p_c"
  Mux5/1 -> Demux6/1, To File1/1
  Pulse Generator/1 -> Sum10/1
  Sum8/1 -> Switch2/1
  LQR/2(Vs) -> Conversion1/2(Vs [V]), Mux8/1
  Demux3/6 -> LQR/5(e_dot)  "e~dot"
  Heli 3D1/6(Elevation rate [rad/s]) -> Mux4/6  "e_dot~"
  Joystick1/2(Y) -> Manual Switch7/1  "e_dot_c"
  Demux3/3 -> LQR/3(p)  "p~"
  Constant7/1 -> Switch1/3
  Constant9/1 -> Sum8/2
  Demux3/4 -> LQR/4(p_dot)  "p~dot"
  Heli 3D1/5(Elevation [rad]) -> Mux4/5  "e~"
  Heli 3D1/2(Travel rate [rad/s]) -> Mux4/2  "lambda_dot~"
  Sum10/1 -> Switch1/1
  Manual Switch5/1 -> Sum6/1
  Mux4/1 -> Estimates/Encoder/2, Mux5/4  "Observer"
  Joystick1/1(X) -> Manual Switch6/2  "p_c"
  Conversion1/2(Vb [V]) -> Heli 3D1/2(Vb [V])
  Demux7/1 -> Observer1/6(V_d)
  Constant5/1 -> Manual Switch5/1
  LQR/1(Vd) -> Conversion1/1(Vd [V]), Mux8/2
  Mux3/1 -> Estimates/Encoder/1, Mux5/5  "Estimates"
  Conversion1/1(Vf [V]) -> Heli 3D1/1(Vf [V])
  [e_dot_hat] -> Scope3/6  "e_dot_hat"
  Demux6/18 -> [e]
  Demux6/9 -> [e_tilda]
  Sum7/1 -> Switch2/2
  Ramp4/1 -> Saturation4/1
  Sum6/1 -> Mux5/3, LQR/2(e_dot_c)
  "Accel vector to [pitch, elevation]1"/1(euler_angles) -> Mux6/1, Demux4/1, "Gyro vector to [pitch rate, elevation rate, travle rate]1"/2(euler_angles)
  Switch2/1 -> Manual Switch7/2
  Demux4/2 -> Observer1/2(e)  "e"
  IMU1/2("gyroscope, rad/s") -> "Gyro vector to [pitch rate, elevation rate, travle rate]1"/1(gyro_vec)  "gyro_vec"
  Manual Switch7/1 -> Sum6/2  "e_dot_c"
  Saturation4/1 -> Manual Switch5/2
  [e_dot_tilda] -> Scope4/10  "e_dot_tilda"
  Demux5/3 -> Observer1/5(lambda_dot)  "lambda_dot"
  IMU1/1("accelerometer, m/s^2") -> "Accel vector to [pitch, elevation]1"/1(accel_vec)  "accel_vec"
  Heli 3D1/3(Pitch [rad]) -> Mux4/3  "p~"
  Demux5/2 -> Observer1/4(e_dot)  "e_dot"
  Demux6/20 -> [e_dot]
  "Gyro vector to [pitch rate, elevation rate, travle rate]1"/1(euler_rates) -> Mux6/2, Demux5/1
  Demux6/1 -> [Vf_sat]
  Step5/1 -> Sum7/1
  Demux6/6 -> [lambda_dot_tilda]
  [p_dot] -> Scope4/6  "p_dot"
  Demux5/1 -> Observer1/3(p_dot)  "p_dot"
  Demux6/11 -> [lamdba_hat]
  Demux4/1 -> Observer1/1(p)  "p"
  [p_tilda] -> Scope3/3  "p_tilda"
  Heli 3D1/7(Vf_sat) -> Mux7/1  "Vf_sat"
  Mux8/1 -> Demux7/1
  Demux7/2 -> Observer1/7(V_s)
  Constant8/1 -> Sum10/2
  [e] -> Scope4/9  "e"
  Step6/1 -> Sum7/2
  Mux7/1 -> Mux5/1
  [e_dot_tilda] -> Scope3/5  "e_dot_tilda"
  Demux6/10 -> [e_dot_tilda]
  [lambda_dot] -> Mux2/5  "Vb_sat"
  [e_dot] -> Mux2/4  "Vb_sat"
  [e] -> Mux2/3  "Vb_sat"
  [p_dot] -> Mux2/2  "Vb_sat"
  [p] -> Mux2/1  "Vb_sat"
  Sum11/1 -> PID Controller1/1
  Constant11/1 -> Sum11/1
  Demux3/2 -> Sum11/2  "lambda_dot"
  Constant12/1 -> LQR/1(p_c)

== system heli_q8_final/Lab_1/Conversion ==
  Vd [V] : Inport
  Vs [V] : Inport  Port=2
  Add : Sum  Inputs=-+
  Back gain : Gain  Gain=0.5
  Front gain : Gain  Gain=0.5
  Subtract : Sum
  Vf [V] : Outport
  Vb [V] : Outport  Port=2
  wires:
  Vd [V]/1 -> Subtract/2, Add/1
  Vs [V]/1 -> Subtract/1, Add/2
  Subtract/1 -> Back gain/1
  Back gain/1 -> Vb [V]/1
  Add/1 -> Front gain/1
  Front gain/1 -> Vf [V]/1

== system heli_q8_final/Lab_1/Elevation controller ==
  e~ [rad] : Inport
  e~dot [rad/s] : Inport  Port=2
  e~c [rad] : Inport  Port=3
  Elevation controller : Subsystem
  Sum : Sum  Inputs=-+  InputSameDT=on  SaturateOnIntegerOverflow=on  OutDataTypeStr=Inherit: Same as first input
  Sum1 : Sum  Inputs=|++
  V_s0 : Constant  Value=V_s0
  V~s [V] : Outport  InitialOutput=0
  wires:
  Sum/1 -> Elevation controller/1(e~ [rad])
  Elevation controller/1(V~_s [V]) -> Sum1/1
  e~ [rad]/1 -> Sum/1
  e~dot [rad/s]/1 -> Elevation controller/2(e~_dot [rad/s])
  e~c [rad]/1 -> Sum/2
  Sum1/1 -> V~s [V]/1
  V_s0/1 -> Sum1/2

== system heli_q8_final/Lab_1/Heli 3D ==
  note: Encoder # 0 - measure Travel angle
      | Encoder # 1 - measure Pitch angle
      | Encoder # 2 - measure Elavation angle
  Vf [V] : Inport
  Vb [V] : Inport  Port=2
  Back motor: Saturation : Saturate  UpperLimit=5  LowerLimit=-5
  Elevation Offset : Constant  Value=elevation_offset
  Elevation: Count to rad : Gain  Gain=-2 * pi /4096
  Elevation: Scope [rad/s] : Scope
  Elevation: Scope [rad] : Scope
  Elevation: Transfer Fcn : TransferFcn  Numerator=[50 0]  Denominator=[1 50]
  Front motor: Saturation : Saturate  UpperLimit=5  LowerLimit=-5
  HIL Read Encoder Timebase : quarc_library/Data Acquisition/Generic/Timebases/HIL Read Encoder Timebase  object_name=HIL-1  clock=0  channels=[0:2]  active=on  vector_output=off  data_type_mode=Inherit via back propagation  data_type=double  overflow_mode=Error on overflow  samples_in_buffer=max(ceil(1/qc_get_step_size), 1)
  HIL Write Analog : quarc_library/Data Acquisition/Generic/Immediate I//O/HIL Write Analog  object_name=HIL-1  channels=[0:1]  sample_time=-1  active=off  vector_input=off
  Pitch: Count to rad : Gain  Gain=-2*pi /4096
  Pitch: Scope [rad] : Scope
  Pitch: Transfer Fcn : TransferFcn  Numerator=[50 0]  Denominator=[1 50]
  Ptich rate: Scope [rad/s] : Scope
  Sum : Sum  Inputs=|+-
  Travel rate: Scope [rad/s] : Scope
  Travel: Count to rad : Gain  Gain=2*pi/8192
  Travel: Scope [rad] : Scope
  Travel: Transfer Fcn : TransferFcn  Numerator=[50 0]  Denominator=[1 50]
  Travel [rad] : Outport
  Travel rate [rad/s] : Outport  Port=2
  Pitch [rad] : Outport  Port=3
  Pitch rate [rad/s] : Outport  Port=4
  Elevation [rad] : Outport  Port=5
  Elevation rate [rad/s] : Outport  Port=6
  wires:
  HIL Read Encoder Timebase/1 -> Travel: Count to rad/1
  HIL Read Encoder Timebase/2 -> Pitch: Count to rad/1
  HIL Read Encoder Timebase/3 -> Elevation: Count to rad/1
  Travel: Count to rad/1 -> Travel: Scope [rad]/1, Travel [rad]/1, Travel: Transfer Fcn/1
  Travel: Transfer Fcn/1 -> Travel rate: Scope [rad/s]/1, Travel rate [rad/s]/1
  Pitch: Count to rad/1 -> Pitch: Transfer Fcn/1, Pitch: Scope [rad]/1, Pitch [rad]/1
  Pitch: Transfer Fcn/1 -> Ptich rate: Scope [rad/s]/1, Pitch rate [rad/s]/1
  Elevation: Count to rad/1 -> Sum/1, Elevation: Transfer Fcn/1
  Elevation: Transfer Fcn/1 -> Elevation: Scope [rad/s]/1, Elevation rate [rad/s]/1
  Vf [V]/1 -> Front motor: Saturation/1
  Vb [V]/1 -> Back motor: Saturation/1
  Front motor: Saturation/1 -> HIL Write Analog/1
  Back motor: Saturation/1 -> HIL Write Analog/2
  Sum/1 -> Elevation: Scope [rad]/1, Elevation [rad]/1
  Elevation Offset/1 -> Sum/2

== system heli_q8_final/Lab_1/Joystick ==
  Dead Zone: x : DeadZone  LowerValue=-0.1  UpperValue=0.1  SaturateOnIntegerOverflow=on
  Dead Zone: y : DeadZone  LowerValue=-0.1  UpperValue=0.1  SaturateOnIntegerOverflow=on
  Gain: x : Gain  Gain=10/9
  Gain: y : Gain  Gain=10/9
  Game Controller : quarc_library/Devices/Peripherals/Target/Game Controller  controller=1  buffer_size=12  deadzone=[]  saturation=[]  sample_time=max(qc_get_step_size, 0.01)  auto_center=off  enabled=on
      settings: SourceProductName=QUARC Targets
  Joystick_gain_x : Gain  Gain=Joystick_gain_x
  Joystick_gain_y : Gain  Gain=Joystick_gain_y
  Rate Transition: x : RateTransition
  Rate Transition: y : RateTransition
  Terminator : Terminator
  Terminator1 : Terminator
  Terminator_{1..2,4..7} (6 alike) : Terminator
  X: Scope : Scope
  Y: Scope : Scope
  X : Outport
  Y : Outport  Port=2
  wires:
  Rate Transition: y/1 -> Dead Zone: y/1
  Rate Transition: x/1 -> Dead Zone: x/1
  Game Controller/5 -> Rate Transition: y/1
  Game Controller/4 -> Rate Transition: x/1
  Game Controller/1 -> Terminator_1/1
  Game Controller/2 -> Terminator_2/1
  Game Controller/7 -> Terminator_4/1
  Game Controller/8 -> Terminator_5/1
  Game Controller/9 -> Terminator_6/1
  Game Controller/10 -> Terminator_7/1
  Game Controller/3 -> Terminator1/1
  Game Controller/6 -> Terminator/1
  Dead Zone: x/1 -> Gain: x/1
  Dead Zone: y/1 -> Gain: y/1
  Gain: x/1 -> Joystick_gain_x/1
  Gain: y/1 -> Joystick_gain_y/1
  Joystick_gain_x/1 -> X/1, X: Scope/1
  Joystick_gain_y/1 -> Y: Scope/1, Y/1

== system heli_q8_final/Lab_1/Pitch controller ==
  p~c [rad] : Inport
  p~ [rad] : Inport  Port=2
  p~dot [rad/s] : Inport  Port=3
  Kpd : Gain  Gain=Kpd
  Kpp : Gain  Gain=Kpp
  Sum : Sum  Inputs=+|-
  Sum1 : Sum  Inputs=|+-
  V~d [V] : Outport  InitialOutput=0
  wires:
  p~c [rad]/1 -> Sum/1
  p~ [rad]/1 -> Sum/2
  Sum/1 -> Kpp/1
  p~dot [rad/s]/1 -> Kpd/1
  Kpp/1 -> Sum1/1
  Kpd/1 -> Sum1/2
  Sum1/1 -> V~d [V]/1

== system heli_q8_final/Lab_2/Conversion ==
  Vd [V] : Inport
  Vs [V] : Inport  Port=2
  Add : Sum  Inputs=-+
  Back gain : Gain  Gain=0.5
  Front gain : Gain  Gain=0.5
  Subtract : Sum
  Vf [V] : Outport
  Vb [V] : Outport  Port=2
  wires:
  Vd [V]/1 -> Subtract/2, Add/1
  Vs [V]/1 -> Subtract/1, Add/2
  Subtract/1 -> Back gain/1
  Back gain/1 -> Vb [V]/1
  Add/1 -> Front gain/1
  Front gain/1 -> Vf [V]/1

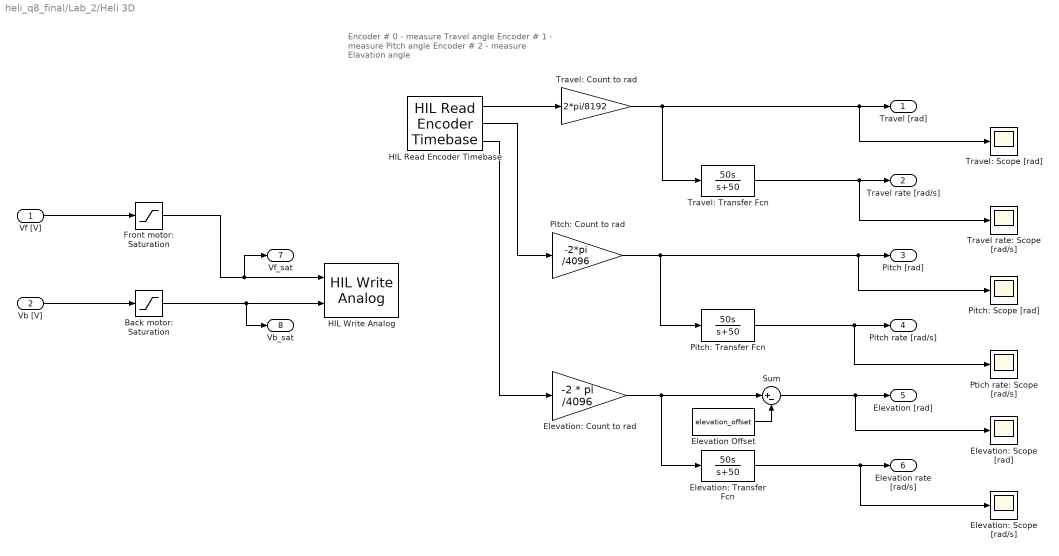
== system heli_q8_final/Lab_2/Heli 3D ==
  note: Encoder # 0 - measure Travel angle
      | Encoder # 1 - measure Pitch angle
      | Encoder # 2 - measure Elavation angle
  Vf [V] : Inport
  Vb [V] : Inport  Port=2
  Back motor: Saturation : Saturate  UpperLimit=5  LowerLimit=-5
  Elevation Offset : Constant  Value=elevation_offset
  Elevation: Count to rad : Gain  Gain=-2 * pi /4096
  Elevation: Scope [rad/s] : Scope
  Elevation: Scope [rad] : Scope
  Elevation: Transfer Fcn : TransferFcn  Numerator=[50 0]  Denominator=[1 50]
  Front motor: Saturation : Saturate  UpperLimit=5  LowerLimit=-5
  HIL Read Encoder Timebase : quarc_library/Data Acquisition/Generic/Timebases/HIL Read Encoder Timebase  object_name=HIL-1  clock=0  channels=[0:2]  active=on  vector_output=off  data_type_mode=Inherit via back propagation  data_type=double  overflow_mode=Error on overflow  samples_in_buffer=max(ceil(1/qc_get_step_size), 1)
  HIL Write Analog : quarc_library/Data Acquisition/Generic/Immediate I//O/HIL Write Analog  object_name=HIL-1  channels=[0:1]  sample_time=-1  active=off  vector_input=off
  Pitch: Count to rad : Gain  Gain=-2*pi /4096
  Pitch: Scope [rad] : Scope
  Pitch: Transfer Fcn : TransferFcn  Numerator=[50 0]  Denominator=[1 50]
  Ptich rate: Scope [rad/s] : Scope
  Sum : Sum  Inputs=|+-
  Travel rate: Scope [rad/s] : Scope
  Travel: Count to rad : Gain  Gain=2*pi/8192
  Travel: Scope [rad] : Scope
  Travel: Transfer Fcn : TransferFcn  Numerator=[50 0]  Denominator=[1 50]
  Travel [rad] : Outport
  Travel rate [rad/s] : Outport  Port=2
  Pitch [rad] : Outport  Port=3
  Pitch rate [rad/s] : Outport  Port=4
  Elevation [rad] : Outport  Port=5
  Elevation rate [rad/s] : Outport  Port=6
  Vf_sat : Outport  Port=7
  Vb_sat : Outport  Port=8
  wires:
  HIL Read Encoder Timebase/1 -> Travel: Count to rad/1
  HIL Read Encoder Timebase/2 -> Pitch: Count to rad/1
  HIL Read Encoder Timebase/3 -> Elevation: Count to rad/1
  Travel: Count to rad/1 -> Travel: Scope [rad]/1, Travel [rad]/1, Travel: Transfer Fcn/1
  Travel: Transfer Fcn/1 -> Travel rate: Scope [rad/s]/1, Travel rate [rad/s]/1
  Pitch: Count to rad/1 -> Pitch: Transfer Fcn/1, Pitch: Scope [rad]/1, Pitch [rad]/1
  Pitch: Transfer Fcn/1 -> Ptich rate: Scope [rad/s]/1, Pitch rate [rad/s]/1
  Elevation: Count to rad/1 -> Sum/1, Elevation: Transfer Fcn/1
  Elevation: Transfer Fcn/1 -> Elevation: Scope [rad/s]/1, Elevation rate [rad/s]/1
  Vf [V]/1 -> Front motor: Saturation/1
  Vb [V]/1 -> Back motor: Saturation/1
  Front motor: Saturation/1 -> HIL Write Analog/1, Vf_sat/1
  Back motor: Saturation/1 -> HIL Write Analog/2, Vb_sat/1
  Sum/1 -> Elevation: Scope [rad]/1, Elevation [rad]/1
  Elevation Offset/1 -> Sum/2

== system heli_q8_final/Lab_2/Joystick ==
  Dead Zone: x : DeadZone  LowerValue=-0.1  UpperValue=0.1  SaturateOnIntegerOverflow=on
  Dead Zone: y : DeadZone  LowerValue=-0.1  UpperValue=0.1  SaturateOnIntegerOverflow=on
  Gain: x : Gain  Gain=10/9
  Gain: y : Gain  Gain=10/9
  Game Controller : quarc_library/Devices/Peripherals/Target/Game Controller  controller=1  buffer_size=12  deadzone=[]  saturation=[]  sample_time=max(qc_get_step_size, 0.01)  auto_center=off  enabled=on
      settings: SourceProductName=QUARC Targets
  Joystick_gain_x : Gain  Gain=Joystick_gain_x
  Joystick_gain_y : Gain  Gain=Joystick_gain_y
  Rate Transition: x : RateTransition
  Rate Transition: y : RateTransition
  Terminator : Terminator
  Terminator1 : Terminator
  Terminator_{1..2,4..7} (6 alike) : Terminator
  X: Scope : Scope
  Y: Scope : Scope
  X : Outport
  Y : Outport  Port=2
  wires:
  Rate Transition: y/1 -> Dead Zone: y/1
  Rate Transition: x/1 -> Dead Zone: x/1
  Game Controller/5 -> Rate Transition: y/1
  Game Controller/4 -> Rate Transition: x/1
  Game Controller/1 -> Terminator_1/1
  Game Controller/2 -> Terminator_2/1
  Game Controller/7 -> Terminator_4/1
  Game Controller/8 -> Terminator_5/1
  Game Controller/9 -> Terminator_6/1
  Game Controller/10 -> Terminator_7/1
  Game Controller/3 -> Terminator1/1
  Game Controller/6 -> Terminator/1
  Dead Zone: x/1 -> Gain: x/1
  Dead Zone: y/1 -> Gain: y/1
  Gain: x/1 -> Joystick_gain_x/1
  Gain: y/1 -> Joystick_gain_y/1
  Joystick_gain_x/1 -> X/1, X: Scope/1
  Joystick_gain_y/1 -> Y: Scope/1, Y/1

== system heli_q8_final/Lab_2/LQR ==
  p_c : Inport
  e_dot_c : Inport  Port=2
  p : Inport  Port=3
  p_dot : Inport  Port=4
  e_dot : Inport  Port=5
  Constant : Constant  Value=V_s0  SampleTime=-1
  Demux : Demux  Outputs=2
  Gain : Gain  Gain=F  Multiplication=Matrix(K*u) (u vector)
  Gain1 : Gain  Gain=K  Multiplication=Matrix(K*u) (u vector)
  Mux : Mux  Inputs=2
  Mux1 : Mux  Inputs=3
  Scope : Scope  NumInputPorts=2
  Scope1 : Scope  NumInputPorts=2
  Sum : Sum  Inputs=|+-
  Sum1 : Sum  Inputs=++|
  Transpose : Math  Operator=transpose  SaturateOnIntegerOverflow=on
  Transpose1 : Math  Operator=transpose  SaturateOnIntegerOverflow=on
  Vd : Outport
  Vs : Outport  Port=2
  wires:
  p_c/1 -> Mux/1
  p/1 -> Mux1/1
  p_dot/1 -> Mux1/2
  e_dot/1 -> Mux1/3
  Mux/1 -> Scope1/1, Transpose/1
  Mux1/1 -> Scope1/2, Transpose1/1
  Gain/1 -> Sum/1
  Gain1/1 -> Sum/2
  Transpose/1 -> Gain/1
  Transpose1/1 -> Gain1/1
  Sum/1 -> Demux/1
  Demux/1 -> Sum1/2, Scope/1  "VS~"
  Constant/1 -> Sum1/1
  Sum1/1 -> Vs/1  "VS"
  e_dot_c/1 -> Mux/2
  Demux/2 -> Scope/2, Vd/1  "VD"

== system heli_q8_final/Lab_2_Integral/Conversion ==
  Vd [V] : Inport
  Vs [V] : Inport  Port=2
  Add : Sum  Inputs=-+
  Back gain : Gain  Gain=0.5
  Front gain : Gain  Gain=0.5
  Subtract : Sum
  Vf [V] : Outport
  Vb [V] : Outport  Port=2
  wires:
  Vd [V]/1 -> Subtract/2, Add/1
  Vs [V]/1 -> Subtract/1, Add/2
  Subtract/1 -> Back gain/1
  Back gain/1 -> Vb [V]/1
  Add/1 -> Front gain/1
  Front gain/1 -> Vf [V]/1

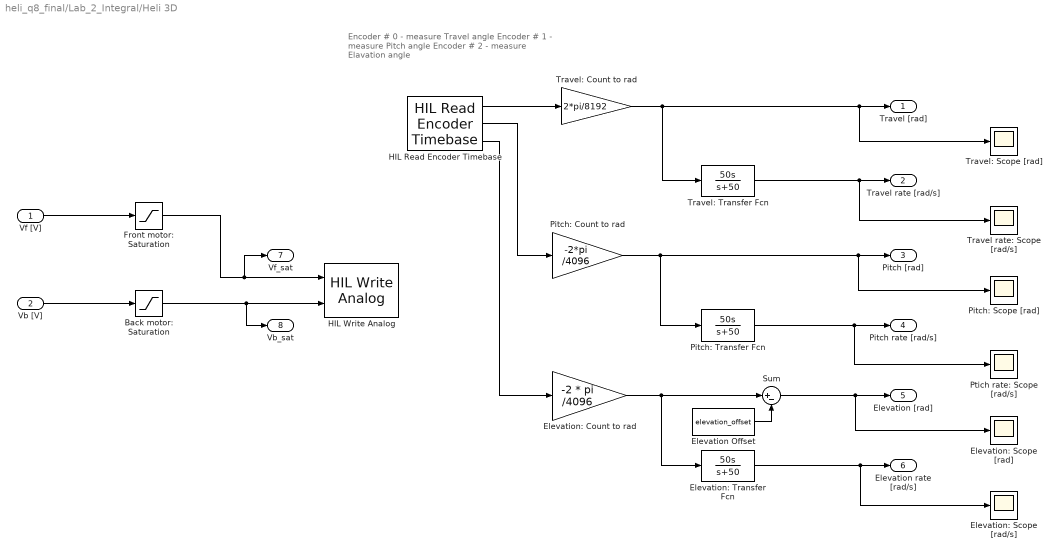
== system heli_q8_final/Lab_2_Integral/Heli 3D ==
  note: Encoder # 0 - measure Travel angle
      | Encoder # 1 - measure Pitch angle
      | Encoder # 2 - measure Elavation angle
  Vf [V] : Inport
  Vb [V] : Inport  Port=2
  Back motor: Saturation : Saturate  UpperLimit=5  LowerLimit=-5
  Elevation Offset : Constant  Value=elevation_offset
  Elevation: Count to rad : Gain  Gain=-2 * pi /4096
  Elevation: Scope [rad/s] : Scope
  Elevation: Scope [rad] : Scope
  Elevation: Transfer Fcn : TransferFcn  Numerator=[50 0]  Denominator=[1 50]
  Front motor: Saturation : Saturate  UpperLimit=5  LowerLimit=-5
  HIL Read Encoder Timebase : quarc_library/Data Acquisition/Generic/Timebases/HIL Read Encoder Timebase  object_name=HIL-1  clock=0  channels=[0:2]  active=on  vector_output=off  data_type_mode=Inherit via back propagation  data_type=double  overflow_mode=Error on overflow  samples_in_buffer=max(ceil(1/qc_get_step_size), 1)
  HIL Write Analog : quarc_library/Data Acquisition/Generic/Immediate I//O/HIL Write Analog  object_name=HIL-1  channels=[0:1]  sample_time=-1  active=off  vector_input=off
  Pitch: Count to rad : Gain  Gain=-2*pi /4096
  Pitch: Scope [rad] : Scope
  Pitch: Transfer Fcn : TransferFcn  Numerator=[50 0]  Denominator=[1 50]
  Ptich rate: Scope [rad/s] : Scope
  Sum : Sum  Inputs=|+-
  Travel rate: Scope [rad/s] : Scope
  Travel: Count to rad : Gain  Gain=2*pi/8192
  Travel: Scope [rad] : Scope
  Travel: Transfer Fcn : TransferFcn  Numerator=[50 0]  Denominator=[1 50]
  Travel [rad] : Outport
  Travel rate [rad/s] : Outport  Port=2
  Pitch [rad] : Outport  Port=3
  Pitch rate [rad/s] : Outport  Port=4
  Elevation [rad] : Outport  Port=5
  Elevation rate [rad/s] : Outport  Port=6
  Vf_sat : Outport  Port=7
  Vb_sat : Outport  Port=8
  wires:
  HIL Read Encoder Timebase/1 -> Travel: Count to rad/1
  HIL Read Encoder Timebase/2 -> Pitch: Count to rad/1
  HIL Read Encoder Timebase/3 -> Elevation: Count to rad/1
  Travel: Count to rad/1 -> Travel: Scope [rad]/1, Travel [rad]/1, Travel: Transfer Fcn/1
  Travel: Transfer Fcn/1 -> Travel rate: Scope [rad/s]/1, Travel rate [rad/s]/1
  Pitch: Count to rad/1 -> Pitch: Transfer Fcn/1, Pitch: Scope [rad]/1, Pitch [rad]/1
  Pitch: Transfer Fcn/1 -> Ptich rate: Scope [rad/s]/1, Pitch rate [rad/s]/1
  Elevation: Count to rad/1 -> Sum/1, Elevation: Transfer Fcn/1
  Elevation: Transfer Fcn/1 -> Elevation: Scope [rad/s]/1, Elevation rate [rad/s]/1
  Vf [V]/1 -> Front motor: Saturation/1
  Vb [V]/1 -> Back motor: Saturation/1
  Front motor: Saturation/1 -> HIL Write Analog/1, Vf_sat/1
  Back motor: Saturation/1 -> HIL Write Analog/2, Vb_sat/1
  Sum/1 -> Elevation: Scope [rad]/1, Elevation [rad]/1
  Elevation Offset/1 -> Sum/2
